simulink model "cooling_fan"  (R2023a)
settings: Solver=FixedStepDiscrete  StartTime=0  StopTime=0.5  FixedStep=0.01  RelTol=1e-3
model workspace (MAT data in the model file):
  CONTROL_PERIOD = 0.1
  FAN_OFF_TEMP = 90
  FAN_ON_TEMP = 95
libraries: simulink x2
settings Model: Creator=sumin  LastModifiedBy=sumin
settings DataIOCC: SaveOutput=off

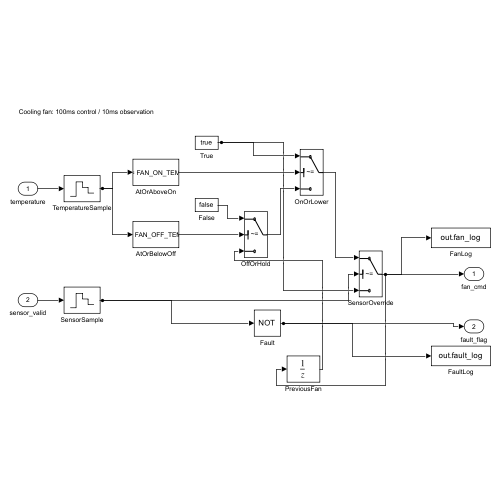
[thumbnail: Simulink's stored preview of the top-level diagram]
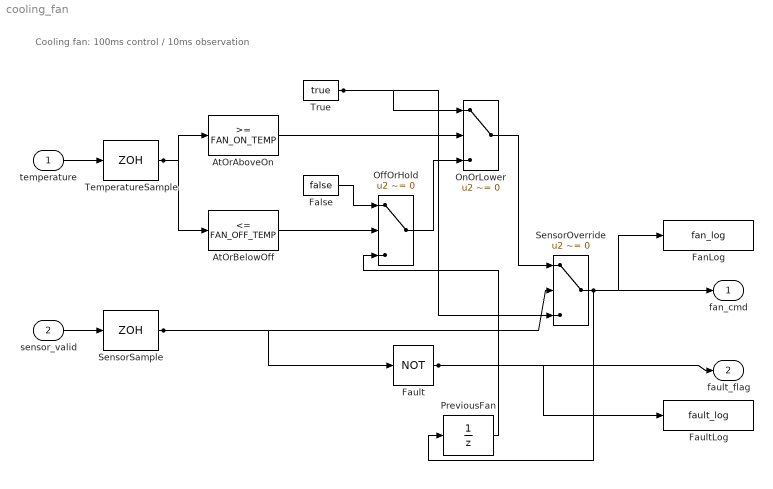
== system cooling_fan ==
  note: Cooling fan: 100ms control / 10ms observation
  temperature : Inport  OutDataTypeStr=double  SampleTime=0.01  Interpolate=off
  sensor_valid : Inport  Port=2  OutDataTypeStr=boolean  SampleTime=0.01  Interpolate=off
  AtOrAboveOn : simulink/Logic and Bit Operations/Compare To Constant  relop=>=  const=FAN_ON_TEMP  OutDataTypeStr=boolean
  AtOrBelowOff : simulink/Logic and Bit Operations/Compare To Constant  relop=<=  const=FAN_OFF_TEMP  OutDataTypeStr=boolean
  False : Constant  Value=false  OutDataTypeStr=boolean
  FanLog : ToWorkspace  VariableName=fan_log  SaveFormat=Timeseries  SampleTime=0.01
  Fault : Logic  Operator=NOT  AllPortsSameDT=off  OutDataTypeStr=boolean
  FaultLog : ToWorkspace  VariableName=fault_log  SaveFormat=Timeseries  SampleTime=0.01
  OffOrHold : Switch  Criteria=u2 ~= 0  SaturateOnIntegerOverflow=off  InputSameDT=off
  OnOrLower : Switch  Criteria=u2 ~= 0  SaturateOnIntegerOverflow=off  InputSameDT=off
  PreviousFan : UnitDelay  InitialCondition=false  SampleTime=CONTROL_PERIOD  HasFrameUpgradeWarning=on
  SensorOverride : Switch  Criteria=u2 ~= 0  SaturateOnIntegerOverflow=off  InputSameDT=off
  SensorSample : ZeroOrderHold  SampleTime=CONTROL_PERIOD
  TemperatureSample : ZeroOrderHold  SampleTime=CONTROL_PERIOD
  True : Constant  Value=true  OutDataTypeStr=boolean
  fan_cmd : Outport
  fault_flag : Outport  Port=2
  wires:
  temperature/1 -> TemperatureSample/1
  sensor_valid/1 -> SensorSample/1
  TemperatureSample/1 -> AtOrAboveOn/1, AtOrBelowOff/1
  False/1 -> OffOrHold/1
  AtOrBelowOff/1 -> OffOrHold/2
  PreviousFan/1 -> OffOrHold/3
  True/1 -> OnOrLower/1, SensorOverride/3
  AtOrAboveOn/1 -> OnOrLower/2
  OffOrHold/1 -> OnOrLower/3
  OnOrLower/1 -> SensorOverride/1
  SensorSample/1 -> SensorOverride/2, Fault/1
  SensorOverride/1 -> PreviousFan/1, fan_cmd/1, FanLog/1
  Fault/1 -> fault_flag/1, FaultLog/1
